simulink model "Drone_simulation_PX4"  (R2025b)
settings: Solver=FixedStepAuto  StartTime=0.0  StopTime=inf  RelTol=1e-6
undefined symbols (not defined in the file): CommParams, fractalcoef, g, Gravity, HIL_GPS_Ts, HIL_HEARTBEAT_Ts, HIL_SENSOR_Ts, HIL_STATE_QUATERNION_Ts, IC, omega_max, Payload, PhysicalScaling, rho_0, SimParams, tau_motor, Tmax_total, Total_mass
libraries: uavmavlinklib x25, slrealtimeiplib x6, sim3dlib x4, aerolibatmos2 x2, matrix_library x1, simulink_extras x1, aerolibasang x1, sensorgpslib x1, mspsensorlib x1, sharedutil x1, aerolibconvert2 x1
(part 2 of 3)

== system Drone_simulation_PX4/TCP // MAVLink Send Subsystem/MAVLink Message Setup/HIL HEARTBEAT ==
  Bus Assignment : BusAssignment  AssignedSignals=Payload.custom_mode,Payload.type,Payload.autopilot,Payload.base_mode,Payload.system_status,Payload.mavlink_version
  Constant : Constant  Value=0  OutDataTypeStr=Inherit: Inherit via back propagation  SampleTime=CommParams.HIL_HEARTBEAT.Ts
  Constant1 : Constant  Value=2  OutDataTypeStr=Inherit: Inherit via back propagation  SampleTime=CommParams.HIL_HEARTBEAT.Ts
  Constant2 : Constant  Value=8  OutDataTypeStr=Inherit: Inherit via back propagation  SampleTime=CommParams.HIL_HEARTBEAT.Ts
  Constant3 : Constant  Value=0  OutDataTypeStr=Inherit: Inherit via back propagation  SampleTime=CommParams.HIL_HEARTBEAT.Ts
  Constant4 : Constant  Value=4  OutDataTypeStr=Inherit: Inherit via back propagation  SampleTime=CommParams.HIL_HEARTBEAT.Ts
  Constant5 : Constant  Value=3  OutDataTypeStr=Inherit: Inherit via back propagation  SampleTime=CommParams.HIL_HEARTBEAT.Ts
  MAVLink Blank Message : uavmavlinklib/MAVLink Blank Message  dialectSource=Select from standard MAVLink dialects  dialect=common.xml  dialectCustom=common.xml  version=2  messageType=HEARTBEAT  SystemID=2  ComponentID=51  SampleTime=CommParams.HIL_HEARTBEAT.Ts
  MAVLink Serializer : uavmavlinklib/MAVLink Serializer  dialectSource=Select from standard MAVLink dialects  dialect=common.xml  dialectCustom=common.xml  version=2  messageType=HEARTBEAT
  Rate Transition : RateTransition  OutPortSampleTime=CommParams.HIL_HEARTBEAT.Ts
  Terminator : Terminator
  HEARTBEAT_DATA : Outport
  wires:
  Constant4/1 -> Bus Assignment/6
  Constant2/1 -> Bus Assignment/4
  MAVLink Blank Message/1 -> Bus Assignment/1
  Constant3/1 -> Bus Assignment/5
  Constant1/1 -> Bus Assignment/3
  Constant/1 -> Bus Assignment/2
  Constant5/1 -> Bus Assignment/7
  Bus Assignment/1 -> Rate Transition/1
  Rate Transition/1 -> MAVLink Serializer/1
  MAVLink Serializer/1 -> HEARTBEAT_DATA/1
  MAVLink Serializer/2 -> Terminator/1

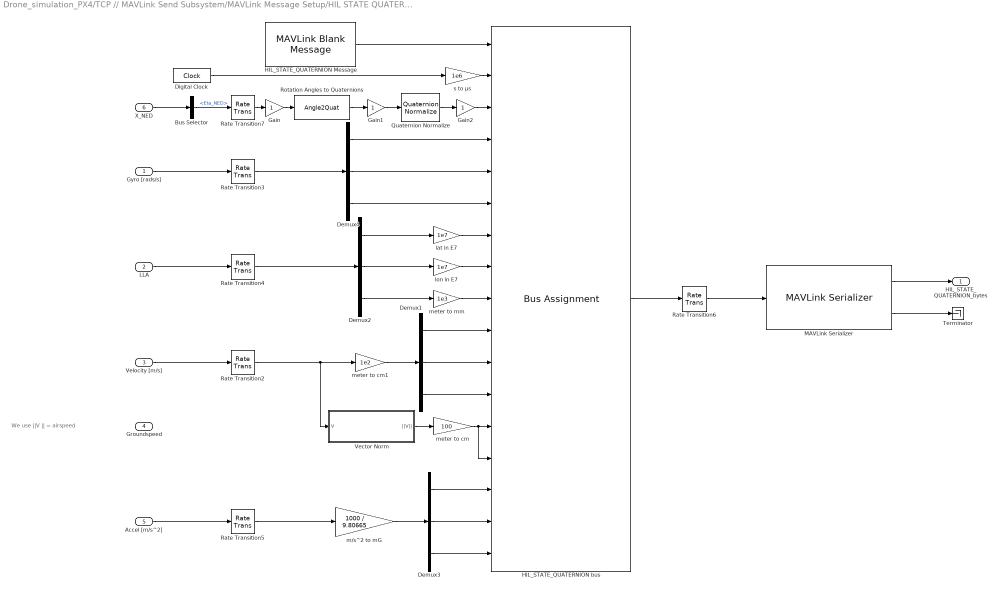
== system Drone_simulation_PX4/TCP // MAVLink Send Subsystem/MAVLink Message Setup/HIL STATE QUATERNION ==
  note: We use ||V || = airspeed
  Gyro [rads/s] : Inport
  LLA : Inport  Port=2
  Velocity [m/s] : Inport  Port=3
  Groundspeed : Inport  Port=4
  Accel [m/s^2] : Inport  Port=5
  X_NED : Inport  Port=6
  Bus Selector : BusSelector  OutputSignals=State.Eta_NED
  Demux{1..4} (4 alike) : Demux  Outputs=3
  Digital Clock : DigitalClock  SampleTime=CommParams.HIL_STATE_QUATERNION.Ts
  Gain : Gain  OutDataTypeStr=Inherit: Inherit via back propagation
  Gain1 : Gain  OutDataTypeStr=Inherit: Inherit via back propagation
  Gain2 : Gain  OutDataTypeStr=Inherit: Inherit via back propagation
  HIL_STATE_QUATERNION Message : uavmavlinklib/MAVLink Blank Message  dialectSource=Select from standard MAVLink dialects  dialect=common.xml  dialectCustom=common.xml  version=2  messageType=HIL_STATE_QUATERNION  SystemID=2  ComponentID=51  SampleTime=-1
  HIL_STATE_QUATERNION bus : BusAssignment  AssignedSignals=Payload.time_usec,Payload.attitude_quaternion,Payload.rollspeed,Payload.pitchspeed,Payload.yawspeed,Payload.lat,Payload.lon,Payload.alt,Payload.vx,Payload.vy,Payload.vz,Payload.ind_airspeed,Payload.true_airspeed,Payload.xacc,Payload.yacc,Payload.zacc
  MAVLink Serializer : uavmavlinklib/MAVLink Serializer  dialectSource=Select from standard MAVLink dialects  dialect=common.xml  dialectCustom=common.xml  version=2  messageType=HIL_STATE_QUATERNION
  Quaternion Normalize : sharedutil/Quaternion Normalize  aMode=aMode
  Rate Transition{2..7} (6 alike) : RateTransition  OutPortSampleTime=CommParams.HIL_STATE_QUATERNION.Ts
  Rotation Angles to Quaternions : Angle2Quat
      settings: AttributesFormatString=Rotation Order: %<rotationOrder>
  Terminator : Terminator
  Vector Norm : Subsystem
  lat in E7 : Gain  Gain=1e7  OutDataTypeStr=int32
  lon in E7 : Gain  Gain=1e7  OutDataTypeStr=int32
  m/s^2 to mG : Gain  Gain=1000 / 9.80665  OutDataTypeStr=int16
  meter to cm : Gain  Gain=100  OutDataTypeStr=Inherit: Inherit via back propagation
  meter to cm1 : Gain  Gain=1e2  OutDataTypeStr=int16
  meter to mm : Gain  Gain=1e3  OutDataTypeStr=int32
  s to µs : Gain  Gain=1e6  OutDataTypeStr=uint64
  HIL_STATE_QUATERNION_bytes : Outport
  wires:
  MAVLink Serializer/1 -> HIL_STATE_QUATERNION_bytes/1
  Rate Transition6/1 -> MAVLink Serializer/1
  HIL_STATE_QUATERNION Message/1 -> HIL_STATE_QUATERNION bus/1
  HIL_STATE_QUATERNION bus/1 -> Rate Transition6/1
  Digital Clock/1 -> s to µs/1
  s to µs/1 -> HIL_STATE_QUATERNION bus/2
  LLA/1 -> Rate Transition4/1
  Demux2/1 -> lat in E7/1
  Demux2/2 -> lon in E7/1
  Demux2/3 -> meter to mm/1
  lat in E7/1 -> HIL_STATE_QUATERNION bus/7
  lon in E7/1 -> HIL_STATE_QUATERNION bus/8
  meter to mm/1 -> HIL_STATE_QUATERNION bus/9
  Velocity [m/s]/1 -> Rate Transition2/1
  Demux1/1 -> HIL_STATE_QUATERNION bus/10
  Demux1/2 -> HIL_STATE_QUATERNION bus/11
  Demux1/3 -> HIL_STATE_QUATERNION bus/12
  meter to cm1/1 -> Demux1/1
  Accel [m/s^2]/1 -> Rate Transition5/1
  m/s^2 to mG/1 -> Demux3/1
  Demux3/1 -> HIL_STATE_QUATERNION bus/15
  Demux3/3 -> HIL_STATE_QUATERNION bus/17
  Gyro [rads/s]/1 -> Rate Transition3/1
  Demux4/1 -> HIL_STATE_QUATERNION bus/4
  Demux4/2 -> HIL_STATE_QUATERNION bus/5
  Demux4/3 -> HIL_STATE_QUATERNION bus/6
  Demux3/2 -> HIL_STATE_QUATERNION bus/16
  Rotation Angles to Quaternions/1 -> Gain1/1
  Quaternion Normalize/1 -> Gain2/1
  Vector Norm/1(||V||) -> meter to cm/1
  meter to cm/1 -> HIL_STATE_QUATERNION bus/14, HIL_STATE_QUATERNION bus/13
  Rate Transition7/1 -> Gain/1
  Gain/1 -> Rotation Angles to Quaternions/1
  Gain1/1 -> Quaternion Normalize/1
  Gain2/1 -> HIL_STATE_QUATERNION bus/3
  X_NED/1 -> Bus Selector/1
  Bus Selector/1 -> Rate Transition7/1  "<Eta_NED>"
  Rate Transition3/1 -> Demux4/1
  Rate Transition4/1 -> Demux2/1
  Rate Transition2/1 -> meter to cm1/1, Vector Norm/1(V)
  Rate Transition5/1 -> m/s^2 to mG/1
  MAVLink Serializer/2 -> Terminator/1

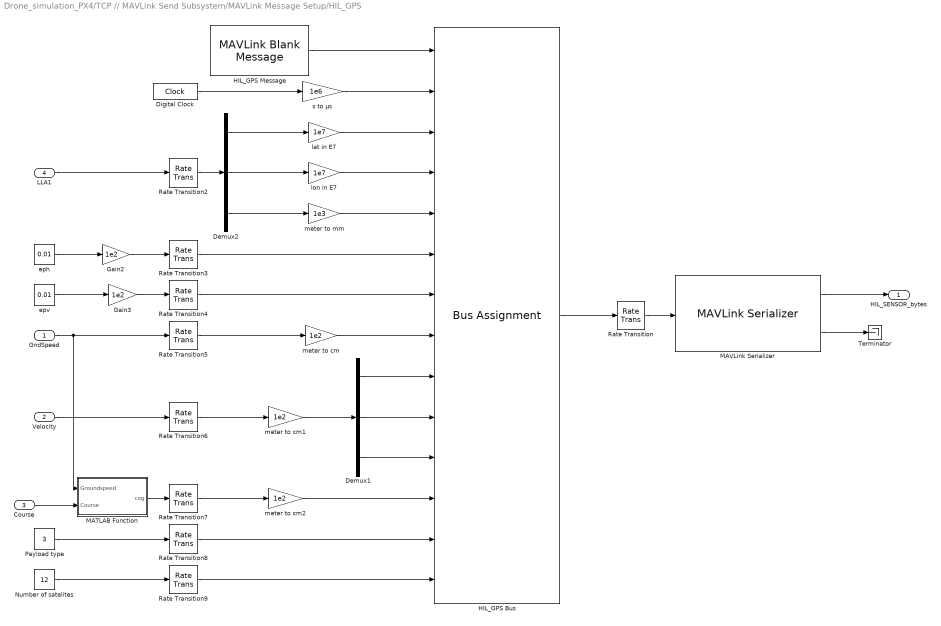
== system Drone_simulation_PX4/TCP // MAVLink Send Subsystem/MAVLink Message Setup/HIL_GPS ==
  GndSpeed : Inport
  Velocity : Inport  Port=2
  Course : Inport  Port=3
  LLA1 : Inport  Port=4
  Demux1 : Demux  Outputs=3
  Demux2 : Demux  Outputs=3
  Digital Clock : DigitalClock  SampleTime=CommParams.HIL_GPS.Ts
  Gain2 : Gain  Gain=1e2  OutDataTypeStr=uint16
  Gain3 : Gain  Gain=1e2  OutDataTypeStr=uint16
  HIL_GPS Bus : BusAssignment  AssignedSignals=Payload.time_usec,Payload.lat,Payload.lon,Payload.alt,Payload.eph,Payload.epv,Payload.vel,Payload.vn,Payload.ve,Payload.vd,Payload.cog,Payload.fix_type,Payload.satellites_visible
  HIL_GPS Message : uavmavlinklib/MAVLink Blank Message  dialectSource=Select from standard MAVLink dialects  dialect=common.xml  dialectCustom=common.xml  version=2  messageType=HIL_GPS  SystemID=2  ComponentID=51  SampleTime=CommParams.HIL_GPS.Ts
  MATLAB Function : MATLAB Function  TreatAsAtomicUnit=on
  MAVLink Serializer : uavmavlinklib/MAVLink Serializer  dialectSource=Select from standard MAVLink dialects  dialect=common.xml  dialectCustom=common.xml  version=2  messageType=HIL_GPS
  Number of satelites : Constant  Value=12  OutDataTypeStr=uint8
  Payload type : Constant  Value=3  OutDataTypeStr=uint8
  Rate Transition{,2..9} (9 alike) : RateTransition  OutPortSampleTime=CommParams.HIL_GPS.Ts
  Terminator : Terminator
  eph : Constant  Value=0.01
  epv : Constant  Value=0.01
  lat in E7 : Gain  Gain=1e7  OutDataTypeStr=int32
  lon in E7 : Gain  Gain=1e7  OutDataTypeStr=int32
  meter to cm : Gain  Gain=1e2  OutDataTypeStr=uint16
  meter to cm1 : Gain  Gain=1e2  OutDataTypeStr=int16
  meter to cm2 : Gain  Gain=1e2  OutDataTypeStr=Inherit: Inherit via back propagation
  meter to mm : Gain  Gain=1e3  OutDataTypeStr=int32
  s to µs : Gain  Gain=1e6  OutDataTypeStr=uint64
  HIL_SENSOR_bytes : Outport
  wires:
  Rate Transition/1 -> MAVLink Serializer/1
  Rate Transition4/1 -> HIL_GPS Bus/7
  Demux2/1 -> lat in E7/1
  s to µs/1 -> HIL_GPS Bus/2
  HIL_GPS Bus/1 -> Rate Transition/1
  meter to cm/1 -> HIL_GPS Bus/8
  Demux1/2 -> HIL_GPS Bus/10
  Rate Transition3/1 -> HIL_GPS Bus/6
  Demux1/1 -> HIL_GPS Bus/9
  Demux1/3 -> HIL_GPS Bus/11
  Number of satelites/1 -> Rate Transition9/1
  GndSpeed/1 -> MATLAB Function/1(Groundspeed), Rate Transition5/1
  Velocity/1 -> Rate Transition6/1
  meter to cm1/1 -> Demux1/1
  Payload type/1 -> Rate Transition8/1
  eph/1 -> Gain2/1
  epv/1 -> Gain3/1
  Digital Clock/1 -> s to µs/1
  lat in E7/1 -> HIL_GPS Bus/3
  lon in E7/1 -> HIL_GPS Bus/4
  meter to mm/1 -> HIL_GPS Bus/5
  LLA1/1 -> Rate Transition2/1
  Demux2/2 -> lon in E7/1
  Demux2/3 -> meter to mm/1
  Rate Transition2/1 -> Demux2/1
  Rate Transition5/1 -> meter to cm/1
  Rate Transition6/1 -> meter to cm1/1
  Rate Transition8/1 -> HIL_GPS Bus/13
  Rate Transition9/1 -> HIL_GPS Bus/14
  MAVLink Serializer/2 -> Terminator/1
  MAVLink Serializer/1 -> HIL_SENSOR_bytes/1
  Rate Transition7/1 -> meter to cm2/1
  Gain2/1 -> Rate Transition3/1
  Gain3/1 -> Rate Transition4/1
  meter to cm2/1 -> HIL_GPS Bus/12
  Course/1 -> MATLAB Function/2(Course)
  MATLAB Function/1(cog) -> Rate Transition7/1
  HIL_GPS Message/1 -> HIL_GPS Bus/1

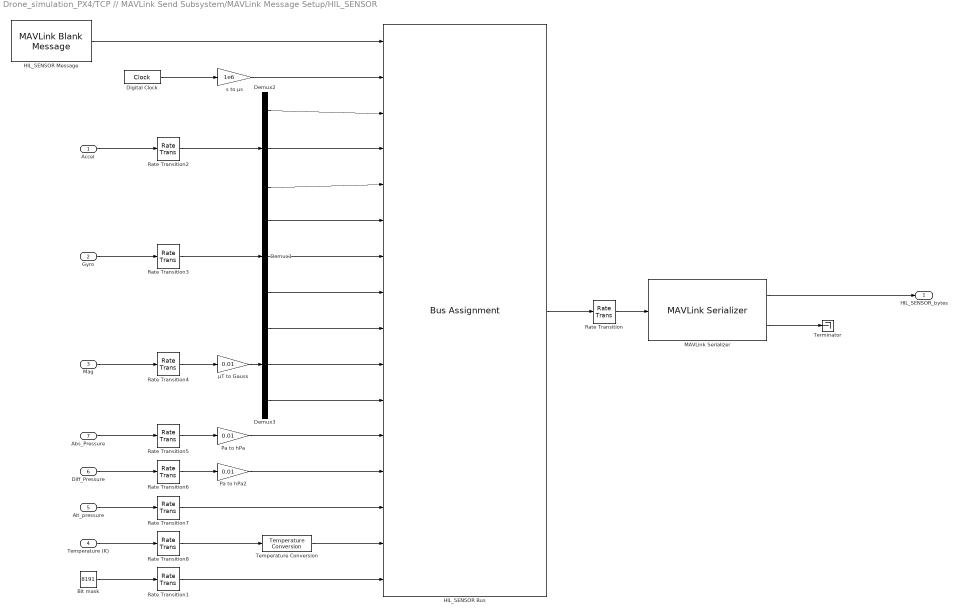
== system Drone_simulation_PX4/TCP // MAVLink Send Subsystem/MAVLink Message Setup/HIL_SENSOR ==
  Accel : Inport
  Gyro : Inport  Port=2
  Mag : Inport  Port=3
  Temperature (K) : Inport  Port=4
  Alt_pressure : Inport  Port=5
  Diff_Pressure : Inport  Port=6
  Abs_Pressure : Inport  Port=7
  Bit mask : Constant  Value=8191  OutDataTypeStr=Inherit: Inherit via back propagation
  Demux1 : Demux  Outputs=3
  Demux2 : Demux  Outputs=3
  Demux3 : Demux  Outputs=3
  Digital Clock : DigitalClock  SampleTime=CommParams.HIL_SENSOR.Ts
  HIL_SENSOR Bus : BusAssignment  AssignedSignals=Payload.time_usec,Payload.xacc,Payload.yacc,Payload.zacc,Payload.xgyro,Payload.ygyro,Payload.zgyro,Payload.xmag,Payload.ymag,Payload.zmag,Payload.abs_pressure,Payload.diff_pressure,Payload.pressure_alt,Payload.temperature,Payload.fields_updated
  HIL_SENSOR Message : uavmavlinklib/MAVLink Blank Message  dialectSource=Select from standard MAVLink dialects  dialect=common.xml  dialectCustom=common.xml  version=2  messageType=HIL_SENSOR  SystemID=2  ComponentID=51  SampleTime=CommParams.HIL_SENSOR.Ts
  MAVLink Serializer : uavmavlinklib/MAVLink Serializer  dialectSource=Select from standard MAVLink dialects  dialect=common.xml  dialectCustom=common.xml  version=2  messageType=HIL_SENSOR
  Pa to hPa : Gain  Gain=0.01  OutDataTypeStr=Inherit: Inherit via back propagation
  Pa to hPa2 : Gain  Gain=0.01  OutDataTypeStr=Inherit: Inherit via back propagation
  Rate Transition{,1..8} (9 alike) : RateTransition  OutPortSampleTime=CommParams.HIL_SENSOR.Ts
  Temperature Conversion : aerolibconvert2/Temperature Conversion  IU=K  OU=C
  Terminator : Terminator
  s to µs : Gain  Gain=1e6  OutDataTypeStr=uint64
  µT to Gauss : Gain  Gain=0.01  OutDataTypeStr=Inherit: Inherit via back propagation
  HIL_SENSOR_bytes : Outport
  wires:
  Rate Transition/1 -> MAVLink Serializer/1
  HIL_SENSOR Message/1 -> HIL_SENSOR Bus/1
  HIL_SENSOR Bus/1 -> Rate Transition/1
  Accel/1 -> Rate Transition2/1
  Demux2/1 -> HIL_SENSOR Bus/3
  Demux2/2 -> HIL_SENSOR Bus/4
  Demux2/3 -> HIL_SENSOR Bus/5
  Demux1/2 -> HIL_SENSOR Bus/7
  Demux1/1 -> HIL_SENSOR Bus/6
  Demux1/3 -> HIL_SENSOR Bus/8
  Gyro/1 -> Rate Transition3/1
  Demux3/1 -> HIL_SENSOR Bus/9
  Demux3/2 -> HIL_SENSOR Bus/10
  Demux3/3 -> HIL_SENSOR Bus/11
  Digital Clock/1 -> s to µs/1
  s to µs/1 -> HIL_SENSOR Bus/2
  µT to Gauss/1 -> Demux3/1
  Mag/1 -> Rate Transition4/1
  Abs_Pressure/1 -> Rate Transition5/1
  Pa to hPa/1 -> HIL_SENSOR Bus/12
  Temperature (K)/1 -> Rate Transition8/1
  Temperature Conversion/1 -> HIL_SENSOR Bus/15
  Alt_pressure/1 -> Rate Transition7/1
  Diff_Pressure/1 -> Rate Transition6/1
  Pa to hPa2/1 -> HIL_SENSOR Bus/13
  Bit mask/1 -> Rate Transition1/1
  Rate Transition2/1 -> Demux2/1
  Rate Transition3/1 -> Demux1/1
  Rate Transition4/1 -> µT to Gauss/1
  Rate Transition5/1 -> Pa to hPa/1
  Rate Transition6/1 -> Pa to hPa2/1
  Rate Transition7/1 -> HIL_SENSOR Bus/14
  Rate Transition8/1 -> Temperature Conversion/1
  MAVLink Serializer/2 -> Terminator/1
  MAVLink Serializer/1 -> HIL_SENSOR_bytes/1
  Rate Transition1/1 -> HIL_SENSOR Bus/16

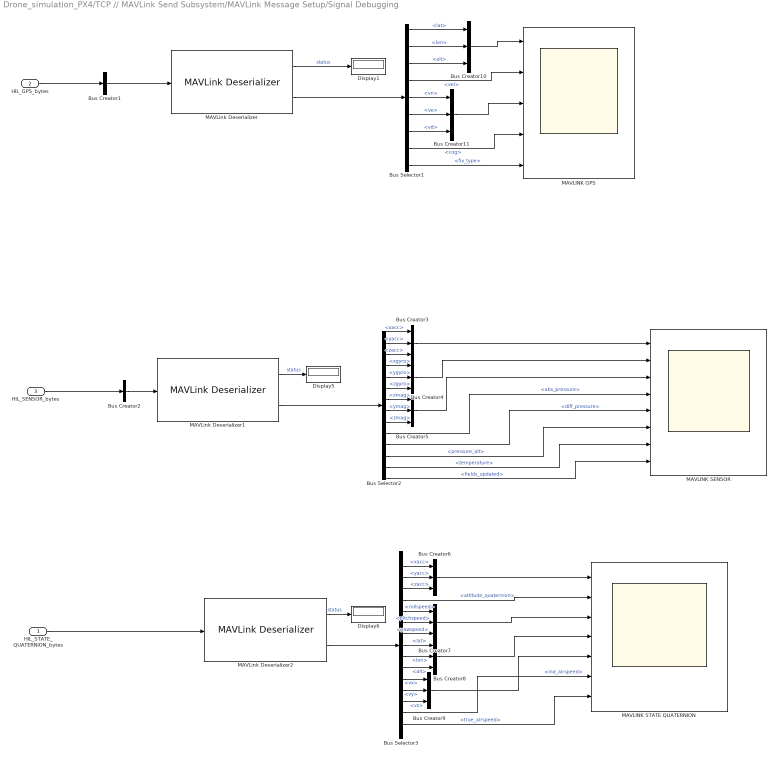
== system Drone_simulation_PX4/TCP // MAVLink Send Subsystem/MAVLink Message Setup/Signal Debugging ==
  HIL_STATE_QUATERNION_bytes : Inport
  HIL_GPS_bytes : Inport  Port=2
  HIL_SENSOR_bytes : Inport  Port=3
  Bus Creator1 : BusCreator  Inputs=1
  Bus Creator{3..11} (9 alike) : BusCreator  Inputs=3
  Bus Creator2 : BusCreator  Inputs=1
  Bus Selector1 : BusSelector  OutputSignals=Payload.lat,Payload.lon,Payload.alt,Payload.vel,Payload.vn,Payload.ve,Payload.vd,Payload.cog,Payload.fix_type
  Bus Selector2 : BusSelector  OutputSignals=Payload.xacc,Payload.yacc,Payload.zacc,Payload.xgyro,Payload.ygyro,Payload.zgyro,Payload.xmag,Payload.ymag,Payload.zmag,Payload.abs_pressure,Payload.diff_pressure,Payload.pressure_alt,Payload.temperature,Payload.fields_updated
  Bus Selector3 : BusSelector  OutputSignals=Payload.xacc,Payload.yacc,Payload.zacc,Payload.attitude_quaternion,Payload.rollspeed,Payload.pitchspeed,Payload.yawspeed,Payload.lat,Payload.lon,Payload.alt,Payload.vx,Payload.vy,Payload.vz,Payload.ind_airspeed,Payload.true_airspeed
  Display1 : Display
  Display5 : Display
  Display6 : Display
  MAVLINK GPS : Scope  NumInputPorts=5
      settings: ActiveDisplayYMinimum=-0.37499999999999989  ActiveDisplayYMaximum=3.375
  MAVLINK SENSOR : Scope  NumInputPorts=8
      settings: ActiveDisplayYMinimum=-0.40522048994898796  ActiveDisplayYMaximum=0.56603492423892021
  MAVLINK STATE QUATERNION : Scope  NumInputPorts=7
      settings: ActiveDisplayYMinimum=-0.088388346135616289  ActiveDisplayYMaximum=0.79549511522054672
  MAVLink Deserializer : uavmavlinklib/MAVLink Deserializer  dialectSource=Select from standard MAVLink dialects  dialect=common.xml  dialectCustom=common.xml  version=2  messageType=HIL_GPS  inputDataLength=off  SystemIDFilter=off  systemID=1  ComponentIDFilter=off  componentID=1  queueMsg=off  queueMsgSize=50  dropNum=off
  MAVLink Deserializer1 : uavmavlinklib/MAVLink Deserializer  dialectSource=Select from standard MAVLink dialects  dialect=common.xml  dialectCustom=common.xml  version=2  messageType=HIL_SENSOR  inputDataLength=off  SystemIDFilter=off  systemID=1  ComponentIDFilter=off  componentID=1  queueMsg=off  queueMsgSize=50  dropNum=off
  MAVLink Deserializer2 : uavmavlinklib/MAVLink Deserializer  dialectSource=Select from standard MAVLink dialects  dialect=common.xml  dialectCustom=common.xml  version=2  messageType=HIL_STATE_QUATERNION  inputDataLength=off  SystemIDFilter=off  systemID=1  ComponentIDFilter=off  componentID=1  queueMsg=off  queueMsgSize=50  dropNum=off
  wires:
  Bus Selector2/10 -> MAVLINK SENSOR/4  "<abs_pressure>"
  Bus Creator1/1 -> MAVLink Deserializer/1
  Bus Selector2/3 -> Bus Creator3/3  "<zacc>"
  Bus Selector1/9 -> MAVLINK GPS/5  "<fix_type>"
  Bus Selector2/4 -> Bus Creator4/1  "<xgyro>"
  Bus Selector2/7 -> Bus Creator5/1  "<xmag>"
  Bus Selector2/6 -> Bus Creator4/3  "<zgyro>"
  MAVLink Deserializer1/1 -> Display5/1  "status"
  Bus Selector1/4 -> MAVLINK GPS/2  "<vel>"
  Bus Selector2/9 -> Bus Creator5/3  "<zmag>"
  Bus Selector1/8 -> MAVLINK GPS/4  "<cog>"
  Bus Selector2/12 -> MAVLINK SENSOR/6  "<pressure_alt>"
  Bus Selector2/11 -> MAVLINK SENSOR/5  "<diff_pressure>"
  MAVLink Deserializer/1 -> Display1/1  "status"
  Bus Selector2/8 -> Bus Creator5/2  "<ymag>"
  Bus Creator3/1 -> MAVLINK SENSOR/1
  Bus Creator4/1 -> MAVLINK SENSOR/2
  MAVLink Deserializer/2 -> Bus Selector1/1
  Bus Creator2/1 -> MAVLink Deserializer1/1
  MAVLink Deserializer1/2 -> Bus Selector2/1
  Bus Creator5/1 -> MAVLINK SENSOR/3
  Bus Selector2/1 -> Bus Creator3/1  "<xacc>"
  Bus Selector2/13 -> MAVLINK SENSOR/7  "<temperature>"
  HIL_GPS_bytes/1 -> Bus Creator1/1
  Bus Selector2/14 -> MAVLINK SENSOR/8  "<fields_updated>"
  Bus Selector2/2 -> Bus Creator3/2  "<yacc>"
  Bus Selector2/5 -> Bus Creator4/2  "<ygyro>"
  HIL_SENSOR_bytes/1 -> Bus Creator2/1
  HIL_STATE_QUATERNION_bytes/1 -> MAVLink Deserializer2/1
  MAVLink Deserializer2/2 -> Bus Selector3/1
  MAVLink Deserializer2/1 -> Display6/1  "status"
  Bus Selector3/1 -> Bus Creator6/1  "<xacc>"
  Bus Selector3/2 -> Bus Creator6/2  "<yacc>"
  Bus Selector3/3 -> Bus Creator6/3  "<zacc>"
  Bus Selector3/5 -> Bus Creator7/1  "<rollspeed>"
  Bus Selector3/6 -> Bus Creator7/2  "<pitchspeed>"
  Bus Selector3/7 -> Bus Creator7/3  "<yawspeed>"
  Bus Selector3/8 -> Bus Creator8/1  "<lat>"
  Bus Selector3/9 -> Bus Creator8/2  "<lon>"
  Bus Selector3/10 -> Bus Creator8/3  "<alt>"
  Bus Selector3/11 -> Bus Creator9/1  "<vx>"
  Bus Selector3/12 -> Bus Creator9/2  "<vy>"
  Bus Selector3/13 -> Bus Creator9/3  "<vz>"
  Bus Selector3/14 -> MAVLINK STATE QUATERNION/6  "<ind_airspeed>"
  Bus Selector3/15 -> MAVLINK STATE QUATERNION/7  "<true_airspeed>"
  Bus Creator6/1 -> MAVLINK STATE QUATERNION/1
  Bus Selector3/4 -> MAVLINK STATE QUATERNION/2  "<attitude_quaternion>"
  Bus Creator7/1 -> MAVLINK STATE QUATERNION/3
  Bus Creator8/1 -> MAVLINK STATE QUATERNION/4
  Bus Creator9/1 -> MAVLINK STATE QUATERNION/5
  Bus Selector1/1 -> Bus Creator10/1  "<lat>"
  Bus Selector1/2 -> Bus Creator10/2  "<lon>"
  Bus Selector1/3 -> Bus Creator10/3  "<alt>"
  Bus Selector1/7 -> Bus Creator11/3  "<vd>"
  Bus Selector1/6 -> Bus Creator11/2  "<ve>"
  Bus Selector1/5 -> Bus Creator11/1  "<vn>"
  Bus Creator11/1 -> MAVLINK GPS/3
  Bus Creator10/1 -> MAVLINK GPS/1

== system Drone_simulation_PX4/Drone Model/Matchematical Drone Model/Drone Dynamics/Mechnical System ==
  note: Dynamical System
  note: Input setup
  Torques and Thurst : Inport
  Bus Creator : BusCreator  Inputs=2
  Bus Creator1 : BusCreator  Inputs=3
  Demux : Demux  Outputs=3
  Demux1 : Demux  Outputs=3
  Rotational Mechanics : Subsystem
      settings: PortSchema="{\"entries\":[{\"content\":{\"sides\":[{\"content\":{\"connectorIds\":[\"In1\",\"In2\",\"In3\"]},\"type\":\"ConnectorPlacement.EquallySpacedRectSide\",\"uuid\":\"0a332066-923f-439e-bae8-eba96ad9ffce\"},{\"content\":{\"connectorIds\":[\"Out1\"],\"side\":\"RIGHT\"},\"type\":\"ConnectorPlacement.EquallySpacedRectSide\",\"uuid\":\"3554fc75-5813-4896-9e16-19d8635f2e75\"},{\"content\":{\"side\":\"TOP\"},\"type\":\"ConnectorPlacement.EquallySpacedRectSide\",\"uuid\":\"32223fd8-6bc7-4616-8423-50c8961bad29\"},{\"content\":{\"connectorIds\":[\"Out2\"],\"side\":\"BOTTOM\"},\"type\":\"ConnectorPlacement.EquallySpacedRectSide\",\"uuid\":\"d3ecfaa1-a069-4309-80f2-d5954d65d4cb\"}]},\"type\":\"ConnectorPlacement.EquallySpacedConnector\",\"uuid\":\"eab4c547-d3d9-4641-a982-ffd3e19f6c7f\"}],\"packageUris\":[\"http://schema.mathworks.com/mf0/Connector/R2020b\"],\"version\":\"1.0\"}"
      mask Display: image('Rotational Mechanics.png');
  Selector : Selector  InputPortWidth=4  IndexOptions=Index vector (dialog)  Indices=[4]  OutputSizes=1
  Selector1 : Selector  InputPortWidth=4  IndexOptions=Index vector (dialog)  Indices=[1 2 3]  OutputSizes=1
  Thrust Saturations : Saturate  UpperLimit=SimParams.MaxTotalThrust  LowerLimit=SimParams.MinTotalThrust
  Torque X Saturations : Saturate  UpperLimit=SimParams.MaxTauX  LowerLimit=SimParams.MinTauX
  Torque Y Saturations : Saturate  UpperLimit=SimParams.MaxTauY  LowerLimit=SimParams.MinTauY
  Torque Z Saturations : Saturate  UpperLimit=SimParams.MaxTauZ  LowerLimit=SimParams.MinTauZ
  "Translational Mechanics " : Subsystem
      settings: PortSchema="{\"entries\":[{\"content\":{\"sides\":[{\"content\":{\"connectorIds\":[\"In1\",\"In2\",\"In3\",\"In4\"]},\"type\":\"ConnectorPlacement.EquallySpacedRectSide\",\"uuid\":\"8c4c4896-0dd8-48ea-87d1-10acad73d291\"},{\"content\":{\"connectorIds\":[\"Out1\",\"Out2\",\"Out3\",\"Out4\"],\"side\":\"RIGHT\"},\"type\":\"ConnectorPlacement.EquallySpacedRectSide\",\"uuid\":\"07a8e31f-79ac-4769-94ea-1ee0808cf567\"},{\"content\":{\"connectorIds\":[\"Out5\"],\"side\":\"TOP\"},\"type\":\"ConnectorPlacement.EquallySpacedRectSide\",\"uuid\":\"0cdf0e6f-f448-460f-b975-01b4b08c4cc5\"}]},\"type\":\"ConnectorPlacement.EquallySpacedConnector\",\"uuid\":\"96a2a48b-dbca-4b5a-a85c-f8caf330b178\"}],\"packageUris\":[\"http://schema.mathworks.com/mf0/Connector/R2020b\"],\"version\":\"1.0\"}"
      mask Display: image('Translational Mechanics.png');
  S [m] : Outport
  S_dot [m/s] : Outport  Port=2
  S_ddot [m/s^2] : Outport  Port=3
  Omega [rads/s] : Outport  Port=4
  Eta [Rads] : Outport  Port=5
  Orientation : Outport  Port=6
  Rho : Outport  Port=7
  Drone inputs : Outport  Port=8
  wires:
  Thrust Saturations/1 -> "Translational Mechanics "/1(Thrust [N]), Bus Creator/1  "Thrust"
  Demux/3 -> "Translational Mechanics "/4(Yaw [Rads])
  Torque Z Saturations/1 -> Rotational Mechanics/3(tau_z [N*m]), Bus Creator1/3  "tau_z"
  Rotational Mechanics/1(Eta [Rads]) -> Eta [Rads]/1, Demux/1  "Eta [Rads]"
  Selector/1 -> Thrust Saturations/1
  Demux1/3 -> Torque Z Saturations/1
  "Translational Mechanics "/2(S_dot [m/s]) -> S_dot [m/s]/1  "S_dot [m/s]"
  Torque X Saturations/1 -> Bus Creator1/1, Rotational Mechanics/1(tau_x [N*m])  "tau_x"
  Torque Y Saturations/1 -> Rotational Mechanics/2(tau_y [N*m]), Bus Creator1/2  "tau_y"
  Demux1/1 -> Torque X Saturations/1
  Demux/2 -> "Translational Mechanics "/3(Pitch [Rads])
  Torques and Thurst/1 -> Selector/1, Selector1/1
  Demux/1 -> "Translational Mechanics "/2(Roll [Rads])
  Selector1/1 -> Demux1/1
  Demux1/2 -> Torque Y Saturations/1
  "Translational Mechanics "/1(S [m]) -> S [m]/1  "S [m]"
  Rotational Mechanics/2(Omega [rads/s]) -> Omega [rads/s]/1  "Omega [rads/s]"
  Bus Creator/1 -> Drone inputs/1
  Bus Creator1/1 -> Bus Creator/2  "Torques"
  "Translational Mechanics "/3(S_ddot [m/s^2]) -> S_ddot [m/s^2]/1  "S_ddot [m/s^2]"
  "Translational Mechanics "/4(Orientation) -> Orientation/1  "Orientation"
  "Translational Mechanics "/5(Rho) -> Rho/1

== system Drone_simulation_PX4/Drone Model/Matchematical Drone Model/Drone Dynamics/Motor Rotor System ==
  Motor CMD : Inport
  Rho : Inport  Port=2
  Legacy Model : Subsystem  Commented=on
  Motor Model : Subsystem
      settings: PortSchema="{\"entries\":[{\"content\":{\"sides\":[{\"content\":{\"connectorIds\":[\"In1\"]},\"type\":\"ConnectorPlacement.EquallySpacedRectSide\",\"uuid\":\"b982dbcd-47b3-4011-8b05-709e276cfd3f\"},{\"content\":{\"connectorIds\":[\"Out1\"],\"side\":\"RIGHT\"},\"type\":\"ConnectorPlacement.EquallySpacedRectSide\",\"uuid\":\"1c27d1a8-dc3d-4e0c-9291-8045ccc685ff\"},{\"content\":{\"side\":\"TOP\"},\"type\":\"ConnectorPlacement.EquallySpacedRectSide\",\"uuid\":\"bc11d3dc-7ca4-46b5-9870-1378c2df1853\"},{\"content\":{\"connectorIds\":[\"Out2\"],\"side\":\"BOTTOM\"},\"type\":\"ConnectorPlacement.EquallySpacedRectSide\",\"uuid\":\"d30f4e93-970d-4e6f-b73c-26678512ef57\"}]},\"type\":\"ConnectorPlacement.EquallySpacedConnector\",\"uuid\":\"a8be81aa-4e4e-4dfa-b42d-c7c42334ef89\"}],\"packageUris\":[\"http://schema.mathworks.com/mf0/Connector/R2020b\"],\"version\":\"1.0\"}"
  Rotor : Subsystem
      settings: PortSchema="{\"entries\":[{\"content\":{\"sides\":[{\"content\":{\"connectorIds\":[\"In1\"]},\"type\":\"ConnectorPlacement.EquallySpacedRectSide\",\"uuid\":\"7759430d-c559-4c9d-9fa2-114d99955e7e\"},{\"content\":{\"connectorIds\":[\"Out1\"],\"side\":\"RIGHT\"},\"type\":\"ConnectorPlacement.EquallySpacedRectSide\",\"uuid\":\"44cff049-b4a7-45db-ae6d-51de1adb222f\"},{\"content\":{\"side\":\"TOP\"},\"type\":\"ConnectorPlacement.EquallySpacedRectSide\",\"uuid\":\"af28e710-9a56-46b8-8f52-f7517d04240a\"},{\"content\":{\"connectorIds\":[\"In2\",\"In3\"],\"side\":\"BOTTOM\"},\"type\":\"ConnectorPlacement.EquallySpacedRectSide\",\"uuid\":\"de596052-a283-4db4-980f-ef32a52a77e8\"}]},\"type\":\"ConnectorPlacement.EquallySpacedConnector\",\"uuid\":\"c454b2a0-97ad-4719-bbb7-f5b86e082541\"}],\"packageUris\":[\"http://schema.mathworks.com/mf0/Connector/R2020b\"],\"version\":\"1.0\"}"
  Drone inputs : Outport
  wires:
  Motor CMD/1 -> Motor Model/1("Motor CMD ")
  Motor Model/1(omega) -> Rotor/1(omega)
  Rho/1 -> Rotor/3(Rho)
  Motor Model/2(omega CMD) -> Rotor/2(omega CMD)
  Rotor/1(u) -> Drone inputs/1

== system Drone_simulation_PX4/TCP // MAVLink Send Subsystem/MAVLink Message Setup/HIL STATE QUATERNION/Vector Norm ==
  V : Inport
  Sqrt : Sqrt
  Square : Math  Operator=square
  Sum of Elements : Sum  Inputs=+
  ||V|| : Outport
  wires:
  V/1 -> Square/1
  Sum of Elements/1 -> Sqrt/1
  Square/1 -> Sum of Elements/1
  Sqrt/1 -> ||V||/1

== system Drone_simulation_PX4/Drone Model/Matchematical Drone Model/Drone Dynamics/Mechnical System/Rotational Mechanics ==
  note: Drag
  tau_x [N*m] : Inport
  tau_y [N*m] : Inport  Port=2
  tau_z [N*m] : Inport  Port=3
  Constant : Constant  Value=SimParams.CdRot
  Cross Product : matrix_library/Cross Product
  Demux : Demux  Outputs=3
  Divide : Product  Inputs=/*  Multiplication=Matrix(*)
  Eta : Integrator  InitialCondition=IC.EulerAngles  WrapState=on  ContinuousStateAttributes={'roll', 'pitch', 'yaw'}
  Euler Rate Matrix : MATLAB Function  TreatAsAtomicUnit=on
  Inertia Matrix : Constant  Value=SimParams.Inertia
  MATLAB Function : MATLAB Function  TreatAsAtomicUnit=on
  Mux : Mux  Inputs=3
  Omega : Integrator  InitialCondition=IC.AngularVelocity  ContinuousStateAttributes={'p', 'q', 'r'}
  Product : Product  Multiplication=Matrix(*)
  Product1 : Product  Multiplication=Matrix(*)
  Scope : Scope  Commented=on
      settings: ActiveDisplayYMinimum=-0.019688460510224104  ActiveDisplayYMaximum=0.018951624166220427  DataLoggingVariableName=ScopeData13
  Sum : Sum  Inputs=++-
  Terminator : Terminator
  Eta [Rads] : Outport
  Omega [rads/s] : Outport  Port=2
  wires:
  tau_y [N*m]/1 -> Mux/2  "tau_y [N*m]"
  tau_x [N*m]/1 -> Mux/1  "tau_x [N*m]"
  Sum/1 -> Divide/2
  Eta/1 -> Eta [Rads]/1, Demux/1  "Eta [Rads]"
  tau_z [N*m]/1 -> Mux/3  "tau_z [N*m]"
  Divide/1 -> Omega/1  "Omega_dot [Rads/s^2]"
  Inertia Matrix/1 -> Divide/1, MATLAB Function/2(J), Product/1
  Mux/1 -> Sum/2  "tau [N*m]"
  Demux/1 -> Euler Rate Matrix/1(roll)  "Roll [rads]"
  Euler Rate Matrix/1(Tmat) -> Product1/1
  Demux/3 -> Terminator/1
  Omega/1 -> Cross Product/1, Product/2, Product1/2, Omega [rads/s]/1, MATLAB Function/1(omega)  "Omega [Rads/s]"
  Demux/2 -> Euler Rate Matrix/2(pitch)  "Pitch [rads]"
  Product1/1 -> Eta/1  "Eta_dot [Rads/s]"
  Product/1 -> Cross Product/2
  Cross Product/1 -> Sum/3
  MATLAB Function/1(tau_drag) -> Sum/1, Scope/1
  Constant/1 -> MATLAB Function/3(CdRot)

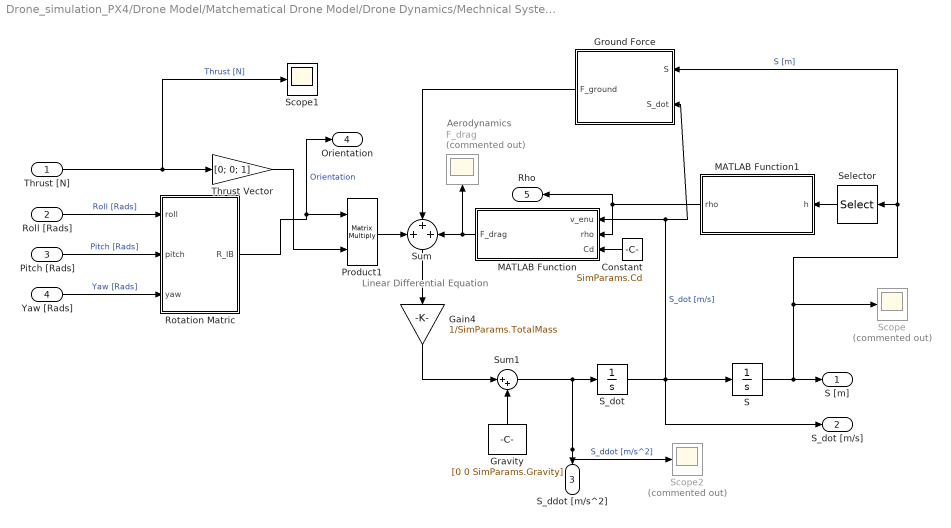
== system Drone_simulation_PX4/Drone Model/Matchematical Drone Model/Drone Dynamics/Mechnical System/Translational Mechanics  ==
  note: Linear Differential Equation
  note: Aerodynamics
  Thrust [N] : Inport
  Roll [Rads] : Inport  Port=2
  Pitch [Rads] : Inport  Port=3
  Yaw [Rads] : Inport  Port=4
  Constant : Constant  Value=SimParams.Cd
  F_drag : Scope  Commented=on
      settings: ActiveDisplayYMinimum=-13.687001257265626  ActiveDisplayYMaximum=2.0306254357297706  DataLoggingVariableName=ScopeData14
  Gain4 : Gain  Gain=1/SimParams.TotalMass
  Gravity : Constant  Value=[0 0 SimParams.Gravity]
  Ground Force : MATLAB Function  TreatAsAtomicUnit=on
  MATLAB Function : MATLAB Function  TreatAsAtomicUnit=on
  MATLAB Function1 : MATLAB Function  TreatAsAtomicUnit=on
  Product1 : Product  Multiplication=Matrix(*)
  Rotation Matric : MATLAB Function  TreatAsAtomicUnit=on
  S : Integrator  InitialCondition=IC.Position  ContinuousStateAttributes={'x', 'y', 'z'}
  S_dot : Integrator  InitialCondition=IC.Velocity  ContinuousStateAttributes={'u', 'v', 'w'}
  Scope : Scope  Commented=on
      settings: ActiveDisplayYMinimum=-1  ActiveDisplayYMaximum=1  DataLoggingVariableName=ScopeData2
  Scope1 : Scope
      settings: ActiveDisplayYMinimum=-1  ActiveDisplayYMaximum=1  DataLoggingVariableName=ScopeData4
  Scope2 : Scope  Commented=on
      settings: DataLoggingVariableName=ScopeData7
  Selector : Selector  InputPortWidth=3  IndexOptions=Index vector (dialog)  Indices=[3]  OutputSizes=1
  Sum : Sum  Inputs=+++
  Sum1 : Sum  Inputs=|++
  Thrust Vector : Gain  Gain=[0; 0; 1]
  S [m] : Outport
  S_dot [m/s] : Outport  Port=2
  S_ddot [m/s^2] : Outport  Port=3
  Orientation : Outport  Port=4
  Rho : Outport  Port=5
  wires:
  Gravity/1 -> Sum1/2
  Rotation Matric/1(R_IB) -> Orientation/1, Product1/1  "Orientation"
  S_dot/1 -> Ground Force/2(S_dot), MATLAB Function/1(v_enu), S/1, S_dot [m/s]/1  "S_dot [m/s]"
  S/1 -> Ground Force/1(S), Selector/1, Scope/1, S [m]/1  "S [m]"
  Gain4/1 -> Sum1/1
  Pitch [Rads]/1 -> Rotation Matric/2(pitch)  "Pitch [Rads]"
  Sum/1 -> Gain4/1
  Roll [Rads]/1 -> Rotation Matric/1(roll)  "Roll [Rads]"
  Thrust [N]/1 -> Scope1/1, Thrust Vector/1  "Thrust [N]"
  Product1/1 -> Sum/1
  Yaw [Rads]/1 -> Rotation Matric/3(yaw)  "Yaw [Rads]"
  Sum1/1 -> Scope2/1, S_ddot [m/s^2]/1, S_dot/1  "S_ddot [m/s^2]"
  Thrust Vector/1 -> Product1/2
  Ground Force/1(F_ground) -> Sum/2
  MATLAB Function/1(F_drag) -> F_drag/1, Sum/3
  Selector/1 -> MATLAB Function1/1(h)
  Constant/1 -> MATLAB Function/3(Cd)
  MATLAB Function1/1(rho) -> Rho/1, MATLAB Function/2(rho)

== system Drone_simulation_PX4/Drone Model/Matchematical Drone Model/Drone Dynamics/Motor Rotor System/Legacy Model ==
  note: Motor Dynamics
  Rho1 : Inport
  In2 : Inport  Port=2
  Display1 : Display  Commented=on
  Gain2 : Gain  Commented=on  Gain=1/rho_0
  Gain3 : Gain  Gain=1/tau_motor
  Integrator1 : Integrator
  MatrixMultiply1 : Product  Commented=on  Multiplication=Matrix(*)
  MatrixMultiply3 : Product  Commented=on  Multiplication=Matrix(*)
  Mixer Matrix1 : Constant  Commented=on  Value="[-1 1 -1 1; -1 -1  1 1; -1 1 1 -1; 1 1 1 1]"
  Omega_max1 : Gain  Gain=omega_max  OutDataTypeStr=Inherit: Inherit via back propagation
  Physical Scaling1 : Constant  Commented=on  Value=PhysicalScaling
  Product1 : Product  Commented=on
  Reshape1 : Reshape  OutputDimensionality=Customize  OutputDimensions=[4,1]
  Selector2 : Selector  Commented=on  InputPortWidth=4  IndexOptions=Index vector (dialog)  Indices=[1 2 3]  OutputSizes=1
  Selector3 : Selector  Commented=on  InputPortWidth=4  IndexOptions=Index vector (dialog)  Indices=[4]  OutputSizes=1
  Square1 : Math  Commented=on  Operator=square
  Sum1 : Sum  Inputs=|+-
  Torques : Outport
  Thrust : Outport  Port=2
  wires:
  MatrixMultiply1/1 -> Selector2/1, Selector3/1
  Omega_max1/1 -> Sum1/1  "omega CMD"
  Product1/1 -> MatrixMultiply1/2
  In2/1 -> Reshape1/1
  Gain3/1 -> Integrator1/1
  Sum1/1 -> Gain3/1
  Integrator1/1 -> Sum1/2, Square1/1  "omega"
  Selector2/1 -> Torques/1  "Torques"
  Square1/1 -> Gain2/1
  Gain2/1 -> Product1/2
  Physical Scaling1/1 -> MatrixMultiply3/1
  Reshape1/1 -> Omega_max1/1
  Rho1/1 -> Product1/1
  Mixer Matrix1/1 -> MatrixMultiply3/2
  MatrixMultiply3/1 -> Display1/1, MatrixMultiply1/1
  Selector3/1 -> Thrust/1  "Thrust"

== system Drone_simulation_PX4/Drone Model/Matchematical Drone Model/Drone Dynamics/Motor Rotor System/Motor Model ==
  note: Motor Dynamics
  "Motor CMD " : Inport
  Gain1 : Gain  Gain=1/SimParams.MotorTimeConstant
  Integrator : Integrator
  Omega_max : Gain  Gain=SimParams.MaxOmega  OutDataTypeStr=Inherit: Inherit via back propagation
  Reshape : Reshape  OutputDimensionality=Customize  OutputDimensions=[4,1]
  Scope : Scope  Commented=on  NumInputPorts=2
      settings: ActiveDisplayYMinimum=-87.336280822753892  ActiveDisplayYMaximum=786.02652740478516  DataLoggingVariableName=ScopeData11
  Sum : Sum  Inputs=|+-
  omega : Outport
  omega CMD : Outport  Port=2
  wires:
  Integrator/1 -> Scope/2, omega/1, Sum/2  "omega"
  Gain1/1 -> Integrator/1
  Reshape/1 -> Omega_max/1
  Omega_max/1 -> Scope/1, Sum/1, omega CMD/1  "omega CMD"
  Sum/1 -> Gain1/1
  "Motor CMD "/1 -> Reshape/1

== system Drone_simulation_PX4/Drone Model/Matchematical Drone Model/Drone Dynamics/Motor Rotor System/Rotor ==
  omega : Inport
  omega CMD : Inport  Port=2
  Rho : Inport  Port=3
  Data Type Conversion : DataTypeConversion  SaturateOnIntegerOverflow=off  RndMeth=Floor
  MATLAB Function : MATLAB Function  TreatAsAtomicUnit=on
  MATLAB Function1 : MATLAB Function  TreatAsAtomicUnit=on
  MultiRotor Scope : Scope  NumInputPorts=4
      settings: ActiveDisplayString=4  ActiveDisplayYMinimum=-0.012633365991743053  ActiveDisplayYMaximum=0.11370029392568751  DataLoggingVariableName=ScopeData16
  Multirotor : Multirotor  armLength=SimParams.ArmLength  rotorHeight=SimParams.RotorHeight  CT=SimParams.CT  CQ=SimParams.CQ  radius=SimParams.RotorRadius
  u : Outport
  wires:
  Multirotor/2 -> MATLAB Function1/2(Mxyz), MultiRotor Scope/4  "Multirotor Torque"
  Data Type Conversion/1 -> MATLAB Function/1(omega)
  MATLAB Function/1(Omega_MW) -> MultiRotor Scope/2, Multirotor/1  "Motor order"
  Multirotor/1 -> MultiRotor Scope/3, MATLAB Function1/1(Fxyz)  "Multirotor Force"
  MATLAB Function1/1(u) -> u/1
  Rho/1 -> Multirotor/2
  omega CMD/1 -> MultiRotor Scope/1  "Omega CMD"
  omega/1 -> Data Type Conversion/1

== matlab function Drone_simulation_PX4/Debugger/TCP // MAVLink Send Subsystem1/HIL_SENSOR/MATLAB Function ==
  data: xacc output; yacc output; zacc output; xgyro output; ygyro output; zgyro output; xmag output; ymag output; zmag output; abs_pressure output; diff_pressure output; pressure_alt output; temperature output; fields_updated output
function [xacc, yacc, zacc, ...
          xgyro, ygyro, zgyro, ...
          xmag, ymag, zmag, ...
          abs_pressure, diff_pressure, pressure_alt, temperature, ...
          fields_updated] = fixed_hil_sensor()
%#codegen
% Fixed HIL_SENSOR for PX4 diagnostic.
%
% MAVLink HIL_SENSOR units:
% accel:         [m/s^2]
% gyro:          [rad/s]
% mag:           [Gauss]
% abs_pressure:  [hPa]
% diff_pressure: [hPa]
% pressure_alt:  [m]
% temperature:   [degC]

% ---------------------------------------------------------
% Fixed level-hover IMU values
% ---------------------------------------------------------

% Accelerometer specific force in PX4 FRD/body convention.
% Level hover should be approximately [0, 0, -g].
xacc = single(0.0);
yacc = single(0.0);
zacc = single(-9.80665);

% Gyroscope body rates
xgyro = single(0.0);
ygyro = single(0.0);
zgyro = single(0.0);

% Magnetometer, fixed reasonable magnetic field [Gauss]
xmag = single(0.27);
ymag = single(-0.03);
zmag = single(-0.16);

% ---------------------------------------------------------
% Barometer
% ---------------------------------------------------------

% Reference altitude 50 m + hover 1 m
alt_m = 51.0;

% Approximate standard-atmosphere pressure at 51 m altitude [hPa]
abs_pressure = single(1013.25 * (1.0 - 2.25577e-5 * alt_m)^5.25588);

diff_pressure = single(0.0);
pressure_alt  = single(alt_m);

temperature = single(15.0);

% Bitmask: all standard fields updated
fields_updated = uint32(8191);

end

== matlab function Drone_simulation_PX4/Drone Model/Matchematical Drone Model/Drone Dynamics/Mechnical System/Translational Mechanics /MATLAB Function ==
  data: v_enu input; F_drag output; rho input; Cd input
function F_drag = aerodynamic_dragGA(v_enu, rho, Cd)
%#codegen
% Quadratic aerodynamic drag in the ENU inertial frame.
%
% Inputs:
%   v_enu : [3x1] velocity relative to air [m/s]
%   rho   : scalar air density [kg/m^3]
%   Cd    : 3-element aerodynamic drag vector [x y z]
%
% Output:
%   F_drag : [3x1] aerodynamic drag force [N]

%% Ensure correct dimensions

v = reshape(single(v_enu), 3, 1);

Cd = reshape(single(Cd), 3, 1);

rho = single(rho);


%% Signed quadratic velocity

v_squared_signed = ...
    abs(v) .* v;


%% Aerodynamic drag force

F_drag = ...
    -single(0.5) .* rho .* Cd .* v_squared_signed;

end

== matlab function Drone_simulation_PX4/Debugger/TCP // MAVLink Send Subsystem1/HIL_GPS/MATLAB Function ==
  data: lat output; lon output; alt output; eph output; epv output; vel output; vn output; ve output; vd output; cog output; fix_type output; satellites_visible output
function [lat, lon, alt, eph, epv, vel, vn, ve, vd, cog, fix_type, satellites_visible] = fixed_gps()
%#codegen

lat0_deg = 55.785;
lon0_deg = 12.521;

alt_m = 51.0;

lat = int32(lat0_deg * 1e7);
lon = int32(lon0_deg * 1e7);
alt = int32(alt_m * 1000);

eph = uint16(100);
epv = uint16(100);

vel = uint16(0);
vn  = int16(0);
ve  = int16(0);
vd  = int16(0);

cog = uint16(65535);

fix_type = uint8(3);
satellites_visible = uint8(10);

end

== matlab function Drone_simulation_PX4/Debugger/MATLAB Function1 ==
  data: t input; m output; test_id input
function m = motor_test_commands(t, test_id)
%#codegen
% Output:
%   m = [m1 m2 m3 m4], single, size 1x4

u_hover = single(0.31243);
d       = single(0.01);

% Explicit fixed-size single output
m = single([u_hover, u_hover, u_hover, u_hover]);

% Convert the Constant-block input to a known integer type
id = uint8(test_id);

if t >= 18.0 && t < 18.2

    switch id
        case uint8(1)
            % Roll: left motors stronger, right motors weaker
            delta = single([-1, 1, -1, 1]);

        case uint8(2)
            % Pitch: rear motors stronger, front motors weaker
            delta = single([-1, -1, 1, 1]);

        case uint8(3)
            % Yaw: motors 1 and 4 stronger
            delta = single([1, -1, -1, 1]);

        otherwise
            delta = single([0, 0, 0, 0]);
    end

    m = m + d .* delta;
end

% Saturate motor commands to [0,1]
m = min(max(m, single(0)), single(1));

end

== matlab function Drone_simulation_PX4/Debugger/MATLAB Function2 ==
  settings: updateMethod=DISCRETE
  data: ready input; u_plant output; u_px4 input; T_hover input
function u_plant = px4_handover(ready, u_px4, T_hover)
%#codegen

persistent alpha

if isempty(alpha)
    alpha = single(0);
end

Ts        = single(0.004);
ramp_time = single(5.0);

u_hover   = [single(0), single(0), single(0), single(T_hover)];
u_px4_row = reshape(single(u_px4), 1, 4);

if ready ~= 0
    alpha = min(alpha + Ts/ramp_time, single(1));
else
    alpha = single(0);
end

u_plant = (single(1) - alpha).*u_hover + alpha.*u_px4_row;

end

== matlab function Drone_simulation_PX4/TCP // MAVLink Send Subsystem/MAVLink Message Setup/HIL_GPS/MATLAB Function ==
  data: Groundspeed input; cog output; Course input
function cog = gps_course_to_cog(Groundspeed, Course)
%#codegen
% Converts GNSS course [deg] to MAVLink HIL_GPS cog [centidegrees].
% If groundspeed is too low, course is undefined, so send 65535.

Groundspeed = single(Groundspeed);
Course = single(Course);

if Groundspeed < single(0.1)
    cog = uint16(65535);
else
    course_deg = Course;

    % Wrap course to [0, 360)
    while course_deg < single(0)
        course_deg = course_deg + single(360);
    end

    while course_deg >= single(360)
        course_deg = course_deg - single(360);
    end

    cog = uint16(course_deg * single(100));
end

end

== matlab function Drone_simulation_PX4/Drone Model/Matchematical Drone Model/Drone Dynamics/MATLAB Function ==
  settings: updateMethod=DISCRETE
  data: u_plant output; u_px4 input; T_motor output; Q_motor output; omega_motor output; rho input
function [u_plant, T_motor, Q_motor, omega_motor] = ...
    motor_propeller_model(u_px4, rho)
%#codegen
% ESC, motor, propeller and air-density model.
%
% Inputs:
%   u_px4 : PX4 motor commands [M1; M2; M3; M4], normalized [0,1]
%   rho   : air density [kg/m^3]
%
% Motor order:
%   M1 = front-right
%   M2 = front-left
%   M3 = rear-right
%   M4 = rear-left
%
% Outputs:
%   u_plant = [tau_x; tau_y; tau_z; total_thrust]
%   T_motor = individual rotor thrusts [N]
%   Q_motor = individual signed yaw moments [N*m]
%   omega_motor = individual rotor speeds [rad/s]

persistent omega

if isempty(omega)
    omega = zeros(4,1,'single');
end


%% Timing

% This block/subsystem must execute at 0.01 seconds.
Ts = single(0.01);

% Lumped ESC and motor time constant
tau_motor = single(0.05);


%% Motor and propeller parameters

rho_0 = single(1.225);       % Reference air density [kg/m^3]

% Keep the currently validated thrust scaling for this test.
Tmax_motor_SL = single(12.0); % Maximum thrust per motor [N]

k_f = single(6.5e-6);        % Thrust coefficient
k_m = single(1.2e-7);        % Reaction-moment coefficient

lever_x = single(0.0955);     % Pitch moment arm [m]
lever_y = single(0.0955);     % Roll moment arm [m]

% The previous mixer limited yaw authority using a safety factor.
% Set this to 0.30 to reproduce the previous mixer behaviour.
yaw_scale = single(0.30);


%% Validated mixer matrix

% Rows:
%   1: roll combination
%   2: pitch combination
%   3: yaw combination
%   4: collective thrust
M = single([ ...
    -1,  1, -1,  1;
    -1, -1,  1,  1;
    -1,  1,  1, -1;
     1,  1,  1,  1]);


%% Sanitize density

rho = single(rho);

if ~isfinite(rho) || rho <= single(0)
    rho = rho_0;
end

rho = min(max(rho, single(0.05)), single(1.50));

density_ratio = rho / rho_0;


%% Sanitize PX4 commands

u = zeros(4,1,'single');

for i = 1:4

    value = single(u_px4(i));

    if ~isfinite(value)
        value = single(0);
    end

    u(i) = min(max(value, single(0)), single(1));
end


%% PX4 command to desired rotor speed

% PX4 command is treated as normalized thrust:
%
%   T_steady = u*Tmax_motor_SL
%
% Since T = k_f*omega^2:
%
%   omega_command = sqrt(u)*omega_max

omega_max = sqrt(Tmax_motor_SL / k_f);

omega_command = sqrt(u) .* omega_max;


%% ESC and motor dynamics

% Exact discrete solution of:
%
%   tau_motor*domega/dt + omega = omega_command

motor_decay = single(exp(-double(Ts / tau_motor)));

omega = ...
    motor_decay .* omega + ...
    (single(1) - motor_decay) .* omega_command;

omega_motor = omega;


%% Individual rotor thrusts

T_motor = ...
    density_ratio .* ...
    k_f .* ...
    omega.^2;


%% Apply the original mixer to actual rotor thrusts

% This is equivalent to the old implementation:
%
%   M*u -> Tmax_motor -> lever-arm gains
%
% but now each rotor includes motor lag and density effects.

mixed_thrust = M * T_motor;


%% Roll and pitch moments

tau_x = lever_y * mixed_thrust(1);
tau_y = lever_x * mixed_thrust(2);


%% Yaw moment

% Since
%
%   T = k_f*omega^2
%   Q = k_m*omega^2
%
% then
%
%   Q/T = k_m/k_f
%
% yaw_scale = 0.30 reproduces the previous yaw-limit scaling.

yaw_moment_per_thrust = ...
    yaw_scale * (k_m / k_f);

tau_z = ...
    yaw_moment_per_thrust * mixed_thrust(3);


%% Individual signed reaction moments

yaw_sign = single([-1; 1; 1; -1]);

Q_motor = ...
    yaw_moment_per_thrust .* ...
    yaw_sign .* ...
    T_motor;


%% Total thrust

T_total = mixed_thrust(4);


%% Plant input

u_plant = single([ ...
    tau_x;
    tau_y;
    tau_z;
    T_total]);

end

== matlab function Drone_simulation_PX4/Drone Model/Matchematical Drone Model/Drone Dynamics/Motor Rotor System/Rotor/MATLAB Function ==
  data: omega input; Omega_MW output
function Omega_MW = multirotor_order(omega)
%#codegen
%
% Input:
% omega = [M1; M2; M3; M4], positive speed magnitudes
%
% M1 = front-right, CCW
% M2 = front-left,  CW
% M3 = rear-right,  CW
% M4 = rear-left,   CCW

Omega_MW = [ ...
     omega(2); ...   % MW rotor 1 = front-left  = CW
    -omega(1); ...   % MW rotor 2 = front-right = CCW
     omega(3); ...   % MW rotor 3 = rear-right   = CW
    -omega(4)];      % MW rotor 4 = rear-left    = CCW

end

== matlab function Drone_simulation_PX4/Drone Model/Matchematical Drone Model/Drone Dynamics/Mechnical System/Rotational Mechanics/MATLAB Function ==
  data: omega input; tau_drag output; J input; CdRot input
function tau_drag = rotational_drag(omega, J, CdRot)
%#codegen
% Linear rotational aerodynamic damping.
%
% Inputs:
%   omega   Body angular velocity [p; q; r] [rad/s]
%   J       Inertia matrix [kg*m^2]
%   CdRot   Rotational drag scaling [roll pitch yaw]
%
% Output:
%   tau_drag Aerodynamic damping torque [N*m]
%
% CdRot = [1 1 1] preserves the nominal damping.
% CdRot = [0 0 0] disables rotational aerodynamic damping.

omega = single(omega);
J     = single(J);
CdRot = reshape(single(CdRot), 3, 1);

%% Nominal free-decay time constants

tau_roll  = single(1.5);     % [s]
tau_pitch = single(1.5);     % [s]
tau_yaw   = single(2.0);     % [s]

%% Nominal rotational damping

D_omega = diag(single([ ...
    J(1,1)/tau_roll;
    J(2,2)/tau_pitch;
    J(3,3)/tau_yaw]));

%% Apply selected aerodynamic scaling

D_omega = diag(CdRot) * D_omega;

%% Aerodynamic damping torque

tau_drag = -D_omega * omega;

end

== matlab function Drone_simulation_PX4/Drone Model/Matchematical Drone Model/Drone Dynamics/Motor Rotor System/Rotor/MATLAB Function1 ==
  data: Fxyz input; u output; Mxyz input
function u = multirotor_to_plant(Fxyz, Mxyz)
%#codegen

% Aerospace FRD -> existing plant FLU convention

tau_x =  Mxyz(1);
tau_y = -Mxyz(2);
tau_z = -Mxyz(3);

T = -Fxyz(3);

u = [ ...
    tau_x;
    tau_y;
    tau_z;
    T];

end

== matlab function Drone_simulation_PX4/MATLAB Function ==
  data: t input; motor_cmd output
function motor_cmd = motor_roll_test(t)
%#codegen
%
% Motor order:
% M1 = front-right
% M2 = front-left
% M3 = rear-right
% M4 = rear-left

omega_base = single(825);
delta      = single(5);

scale = single(16011);

% Default: approximately hover / slight upward thrust
omega_cmd = single([ ...
    omega_base;
    omega_base;
    omega_base;
    omega_base]);

% Small positive-roll pulse
if t >= single(2.0) && t < single(2.2)

    omega_cmd = single([ ...
        omega_base - delta;   % M1 = 820
        omega_base + delta;   % M2 = 830
        omega_base - delta;   % M3 = 820
        omega_base + delta]); % M4 = 830
end

motor_cmd = omega_cmd ./ scale;

end

== matlab function Drone_simulation_PX4/Drone Model/Matchematical Drone Model/Drone Dynamics/Mechnical System/Translational Mechanics /MATLAB Function1 ==
  data: h input; rho output
function rho  = isa_atmosphere(h)
%#codegen
% ISA atmosphere model for the troposphere.
%
% Input:
%   h   Altitude above mean sea level [m]
%
% Outputs:
%   T   Temperature [K]
%   a   Speed of sound [m/s]
%   P   Atmospheric pressure [Pa]
%   rho Air density [kg/m^3]

% ISA sea-level constants
T0    = 288.15;       % [K]
P0    = 101325.0;     % [Pa]
g0    = 9.80665;      % [m/s^2]
R_air = 287.05287;    % [J/(kg*K)]
L     = 0.0065;       % [K/m], temperature lapse rate

% Keep the model inside the troposphere validity range
h = min(max(h, -500.0), 11000.0);

% ISA temperature
T = T0 - L*h;

% ISA pressure
P = P0*(T/T0)^(g0/(R_air*L));

% Ideal-gas density
rho = P/(R_air*T);

end
